simulink model "rectifier"  (R2025a)
settings: Solver=VariableStepAuto  StartTime=0.0  StopTime=0.1  RelTol=1e-3
libraries: spsDiodeLib x4, spsVoltageMeasurementLib x2, spsACVoltageSourceLib x1, spsSeriesRLCBranchLib x1, sps_lib x1
settings Model: Creator=aayush  LastModifiedBy=aayush

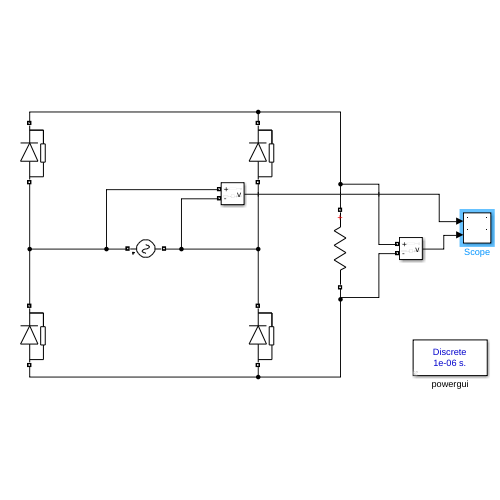
[thumbnail: Simulink's stored preview of the top-level diagram]
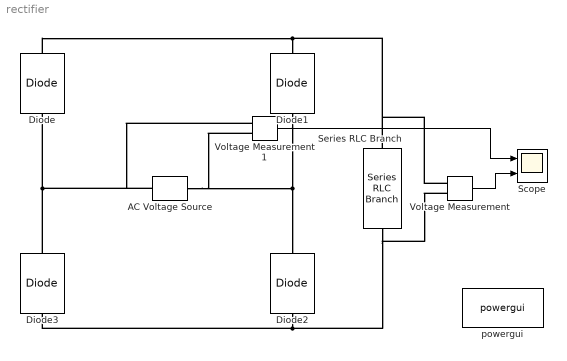
== system rectifier ==
  AC Voltage Source : spsACVoltageSourceLib/AC Voltage Source  Amplitude=230  Phase=0  Frequency=50  SampleTime=0  Measurements=None  BusType=swing  Pref=10e3  Qref=0  Qmin=-inf  Qmax=+inf
  Diode{,1..3} (4 alike) : spsDiodeLib/Diode  Ron=0.001  Lon=0  Vf=0.8  IC=0  UseSnubber=0  Rs=500  Cs=250e-9  Measurements=off
  Scope : Scope  NumInputPorts=2
      settings: ActiveDisplayYMinimum=-287.5  ActiveDisplayYMaximum=287.5
  Series RLC Branch : spsSeriesRLCBranchLib/Series RLC Branch  LConnTagsString=__new0  RConnTagsString=__new0  BranchType=R  Resistance=100  Inductance=1e-3  SetiL0=off  InitialCurrent=0  Capacitance=1e-6  Setx0=off  InitialVoltage=0  Measurements=None
  Voltage Measurement : spsVoltageMeasurementLib/Voltage Measurement  PhasorSimulation=off  OutputType=Complex  PSBequivalent=0
  Voltage Measurement1 : spsVoltageMeasurementLib/Voltage Measurement  PhasorSimulation=off  OutputType=Complex  PSBequivalent=0
  powergui : sps_lib/powergui  Priority=1  SimulationMode=Discrete  SampleTime=1e-6  frequency=50  Iterations=50  frequencyindice=0  Pbase=100e6  ErrMax=1e-4  UnitsV=kV  UnitsW=MW  buscounter=0  FunctionMessages=off  echomessages=off  EnableUseOfTLC=off  CurrentSourceSwitches=off  DisableSnubberDevices=off  DisableRonSwitches=off  DisableVfSwitches=off  DisplayEquations=off  AutomaticDiscreteSolvers=off  SolverType=Tustin/Backward Euler (TBE)  Interpol=off  ExternalGateDelay=off  methode=off  Ts=100  x0status=blocks  SPID=on  SwTol=0  HookPort=off  NonlinearTolerance=1e-4  nMaxIteration=100  ContinueOnMaxIteration=off  RestoreLinks=warning  ResistiveCurrentMeasurement=off  Frange=[0:2:500]  Ylog=off  Xlog=on  ShowGrid=off  save=off  variable=ZData  structure=0  ZoomFFT=off  StartTime=0.0  cycles=1  DisplayStyle=1  fundamental=60  FreqAxis=off  MaxFrequency=1000  frequencyindicesteady=1  RmsSteady=1  display=off
  wires:
  Voltage Measurement/1 -> Scope/2
  Voltage Measurement1/1 -> Scope/1
  connections:
  Diode3/RConn1 -- Voltage Measurement1/LConn1 -- AC Voltage Source/RConn1 -- Diode/LConn1
  Diode1/LConn1 -- Voltage Measurement1/LConn2 -- AC Voltage Source/LConn1 -- Diode2/RConn1
  Diode2/LConn1 -- Voltage Measurement/LConn2 -- Series RLC Branch/RConn1 -- Diode3/LConn1
  Diode/RConn1 -- Voltage Measurement/LConn1 -- Series RLC Branch/LConn1 -- Diode1/RConn1
